simulink model "ecu_relay"  (R2026a)
settings: Solver=FixedStepDiscrete  StopTime=10  FixedStep=0.001  SampleTimeConstraint=STIndependent
Description:
  | Main relay and after-run. Source of truth for firmware/gen/ecu_relay.
settings Model: Creator=jj1001000  LastModifiedBy=jj1001000
settings OptimizationCC: DefaultUnderspecifiedDataType=single
settings DebuggingCC: ParameterPrecisionLossMsg=none
settings HardwareCC: ProdLargestAtomicInteger=Long  ProdLargestAtomicFloat=Double  ProdHWDeviceType=ARM Compatible->ARM Cortex-M
settings RTWCC: SystemTargetFile=ert.tlc  GenCodeOnly=on  Description=Embedded Coder
settings ERTTargetCC: UtilityFuncGeneration=Shared location  IncludeMdlTerminateFcn=off  CodeInterfacePackaging=Reusable function  SupportNonFinite=off

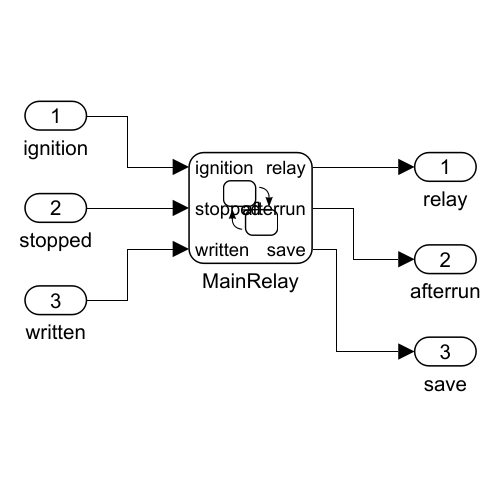
[thumbnail: Simulink's stored preview of the top-level diagram]
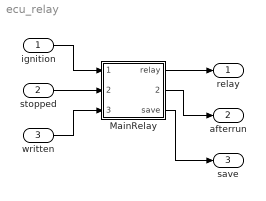
== system ecu_relay ==
  ignition : Inport  OutDataTypeStr=uint8
  stopped : Inport  Port=2  OutDataTypeStr=uint8
  written : Inport  Port=3  OutDataTypeStr=uint8
  MainRelay : Stateflow chart  TreatAsAtomicUnit=on
  relay : Outport  OutDataTypeStr=uint8
  afterrun : Outport  Port=2  OutDataTypeStr=uint8
  save : Outport  Port=3  OutDataTypeStr=uint8
  wires:
  ignition/1 -> MainRelay/1(ignition)
  MainRelay/3(save) -> save/1
  MainRelay/1(relay) -> relay/1
  stopped/1 -> MainRelay/2(stopped)
  MainRelay/2(afterrun) -> afterrun/1
  written/1 -> MainRelay/3(written)

== stateflow chart ecu_relay/MainRelay ==
  settings: updateMethod=DISCRETE  executeAtInitialization=1
  state Relay
    entry: ms = uint16(0); save = uint8(0);
    during: save = uint8(0);
    state AFTER_RUN
      entry: relay = uint8(1); afterrun = uint8(1);
      during: ms = min(ms + 1, uint16(60000));
    state OFF
      entry: relay = uint8(0); afterrun = uint8(0);
    state HELD
      entry: relay = uint8(1); afterrun = uint8(0);
    (default) -> OFF
    HELD -> AFTER_RUN : [ignition == 0]{save = uint8(1); ms = uint16(1);}
    OFF -> HELD : [ignition ~= 0]
    AFTER_RUN -> HELD [order 1] : [ignition ~= 0]{ms = uint16(0);}
    AFTER_RUN -> OFF [order 2] : [(stopped ~= 0 && written ~= 0) || ms + 1 >= uint16(60000)]
  (default) -> Relay
  data: ignition input uint8; stopped input uint8; written input uint8; relay output uint8; afterrun output uint8; save output uint8; ms local uint16
